simulink library "casper_library_correlator"  (Simulink 8.0)
settings: Solver=ode45  SolverMode=SingleTasking  StartTime=0.0  StopTime=10.0  RelTol=1e-3
values from neighbouring files (symbols this model uses):
  n_bits = eval(get_var('n_bits', 'defaults', defaults, varargin{:}))    [auto_tap_init.m]    (also in baseline_tap_init.m; bi_real_unscr_2x_init.m = get_var('n_bits', 'defaults', defaults, varargin{:}); bi_real_unscr_4x_init.m = get_var('n_bits', 'defaults', defaults, varargin{:}); bit_reverse_init.m = get_var('n_bits',varargin{:}))
libraries: xbsIndex_r4 x1360, casper_library_misc x140, casper_library_multipliers x32, xps_library x8, casper_library_delays x1, casper_library_correlator x1
(part 4 of 14)

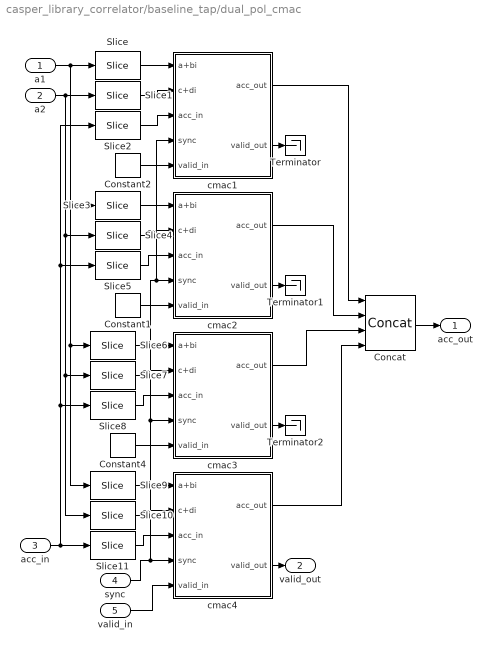
== system casper_library_correlator/baseline_tap/dual_pol_cmac ==
  a1 : Inport
  a2 : Inport  Port=2
  acc_in : Inport  Port=3
  sync : Inport  Port=4
  valid_in : Inport  Port=5
  Concat : xbsIndex_r4/Concat  num_inputs=4  dbl_ovrd=off  block_type=concat
      settings: block_version=9.2.01
  Constant1 : xbsIndex_r4/Constant  const=0  gui_display_data_type=Fixed-point  arith_type=Unsigned  n_bits=1  bin_pt=0  preci_type=Single  exp_width=8  frac_width=24  explicit_period=on  period=1  equ=P=C  opselect=C  inp2=PCIN>>17  opr=+  inp1=P  carry=CIN  dbl_ovrd=off  block_type=constant
      settings: block_version=9.2.01
  Constant2 : xbsIndex_r4/Constant  const=0  gui_display_data_type=Fixed-point  arith_type=Unsigned  n_bits=1  bin_pt=0  preci_type=Single  exp_width=8  frac_width=24  explicit_period=on  period=1  equ=P=C  opselect=C  inp2=PCIN>>17  opr=+  inp1=P  carry=CIN  dbl_ovrd=off  block_type=constant
      settings: block_version=9.2.01
  Constant4 : xbsIndex_r4/Constant  const=0  gui_display_data_type=Fixed-point  arith_type=Unsigned  n_bits=1  bin_pt=0  preci_type=Single  exp_width=8  frac_width=24  explicit_period=on  period=1  equ=P=C  opselect=C  inp2=PCIN>>17  opr=+  inp1=P  carry=CIN  dbl_ovrd=off  block_type=constant
      settings: block_version=9.2.01
  Slice{,1,6,10} (4 alike) : xbsIndex_r4/Slice  nbits=2*n_bits  boolean_output=off  mode=Upper Bit Location + Width  bit1=0  base1=MSB of Input  bit0=0  base0=LSB of Input  dbl_ovrd=off  block_type=slice
      Slice settings: infoedit="Extracts a given range of bits from each input sample and presents it at the output.  The output type is ordinarily unsigned with binary point at zero, but can be Boolean when the slice is one bit wide.<P><P>Hardware notes: In hardware this block costs nothing."  block_version=9.2.01
      Slice1 settings: infoedit="Extracts a given range of bits from each input sample and presents it at the output.  The output type is ordinarily unsigned with binary point at zero, but can be Boolean when the slice is one bit wide.<P><P>Hardware notes: In hardware this block costs nothing."  block_version=9.2.01
      Slice10 settings: block_version=9.2.01
      Slice6 settings: infoedit="Extracts a given range of bits from each input sample and presents it at the output.  The output type is ordinarily unsigned with binary point at zero, but can be Boolean when the slice is one bit wide.<P><P>Hardware notes: In hardware this block costs nothing."  block_version=9.2.01
  Slice11 : xbsIndex_r4/Slice  nbits=2*n_bits_out  boolean_output=off  mode=Upper Bit Location + Width  bit1=-6*n_bits_out  base1=MSB of Input  bit0=0  base0=LSB of Input  dbl_ovrd=off  block_type=slice
      settings: infoedit="Extracts a given range of bits from each input sample and presents it at the output.  The output type is ordinarily unsigned with binary point at zero, but can be Boolean when the slice is one bit wide.<P><P>Hardware notes: In hardware this block costs nothing."  block_version=9.2.01
  Slice2 : xbsIndex_r4/Slice  nbits=2*n_bits_out  boolean_output=off  mode=Upper Bit Location + Width  bit1=0  base1=MSB of Input  bit0=0  base0=LSB of Input  dbl_ovrd=off  block_type=slice
      settings: infoedit="Extracts a given range of bits from each input sample and presents it at the output.  The output type is ordinarily unsigned with binary point at zero, but can be Boolean when the slice is one bit wide.<P><P>Hardware notes: In hardware this block costs nothing."  block_version=9.2.01
  Slice{3..4,7,9} (4 alike) : xbsIndex_r4/Slice  nbits=2*n_bits  boolean_output=off  mode=Upper Bit Location + Width  bit1=-2*n_bits  base1=MSB of Input  bit0=0  base0=LSB of Input  dbl_ovrd=off  block_type=slice
      Slice3 settings: infoedit="Extracts a given range of bits from each input sample and presents it at the output.  The output type is ordinarily unsigned with binary point at zero, but can be Boolean when the slice is one bit wide.<P><P>Hardware notes: In hardware this block costs nothing."  block_version=9.2.01
      Slice4 settings: infoedit="Extracts a given range of bits from each input sample and presents it at the output.  The output type is ordinarily unsigned with binary point at zero, but can be Boolean when the slice is one bit wide.<P><P>Hardware notes: In hardware this block costs nothing."  block_version=9.2.01
      Slice7 settings: infoedit="Extracts a given range of bits from each input sample and presents it at the output.  The output type is ordinarily unsigned with binary point at zero, but can be Boolean when the slice is one bit wide.<P><P>Hardware notes: In hardware this block costs nothing."  block_version=9.2.01
      Slice9 settings: block_version=9.2.01
  Slice5 : xbsIndex_r4/Slice  nbits=2*n_bits_out  boolean_output=off  mode=Upper Bit Location + Width  bit1=-2*n_bits_out  base1=MSB of Input  bit0=0  base0=LSB of Input  dbl_ovrd=off  block_type=slice
      settings: infoedit="Extracts a given range of bits from each input sample and presents it at the output.  The output type is ordinarily unsigned with binary point at zero, but can be Boolean when the slice is one bit wide.<P><P>Hardware notes: In hardware this block costs nothing."  block_version=9.2.01
  Slice8 : xbsIndex_r4/Slice  nbits=2*n_bits_out  boolean_output=off  mode=Upper Bit Location + Width  bit1=-4*n_bits_out  base1=MSB of Input  bit0=0  base0=LSB of Input  dbl_ovrd=off  block_type=slice
      settings: infoedit="Extracts a given range of bits from each input sample and presents it at the output.  The output type is ordinarily unsigned with binary point at zero, but can be Boolean when the slice is one bit wide.<P><P>Hardware notes: In hardware this block costs nothing."  block_version=9.2.01
  Terminator : Terminator
  Terminator1 : Terminator
  Terminator2 : Terminator
  cmac1 : Subsystem  Tag=cmac  AncestorBlock=casper_library_correlator/cmac  mask(cmac){acc_len=128, n_bits_a=4, bin_pt_a=3, n_bits_b=4, bin_pt_b=3, quantization=Truncate, overflow=Wrap, mult_latency=1, add_latency=1, in_latency=0, conv_latency=0, multiplier_implementation=embedded multiplier core}
      mask prompts: acc_len "Number of Accumulations"; n_bits_a "Number of bits 'a'"; bin_pt_a "Binary point 'a'"; n_bits_b "Number of bits 'b'"; bin_pt_b "Binary point 'b'"; quantization "Quantisation"; mult_latency "Multiplier Latency"; add_latency "Adder Latency"; in_latency "Input Latency"; conv_latency "Convert Latency"; multiplier_implementation "Multiplier Implementation"
      mask help: A complex multiply-accumulate block. Full precision.
      mask init: same as casper_library_correlator/dual_pol_cmac/cmac1
      mask TypeOptions quantization: Truncate | Round  (unbiased: +/- Inf) | Round  (unbiased: Even Values)
      mask TypeOptions overflow: Wrap | Saturate | Flag as error
      mask TypeOptions multiplier_implementation: behavioral HDL | standard core | embedded multiplier core
  cmac2 : Subsystem  Tag=cmac  AncestorBlock=casper_library_correlator/cmac  mask(cmac){acc_len=128, n_bits_a=4, bin_pt_a=3, n_bits_b=4, bin_pt_b=3, quantization=Truncate, overflow=Wrap, mult_latency=1, add_latency=1, in_latency=0, conv_latency=0, multiplier_implementation=embedded multiplier core}
      mask prompts: acc_len "Number of Accumulations"; n_bits_a "Number of bits 'a'"; bin_pt_a "Binary point 'a'"; n_bits_b "Number of bits 'b'"; bin_pt_b "Binary point 'b'"; quantization "Quantisation"; mult_latency "Multiplier Latency"; add_latency "Adder Latency"; in_latency "Input Latency"; conv_latency "Convert Latency"; multiplier_implementation "Multiplier Implementation"
      mask help: A complex multiply-accumulate block. Full precision.
      mask init: same as casper_library_correlator/dual_pol_cmac/cmac1
      mask TypeOptions quantization: Truncate | Round  (unbiased: +/- Inf) | Round  (unbiased: Even Values)
      mask TypeOptions overflow: Wrap | Saturate | Flag as error
      mask TypeOptions multiplier_implementation: behavioral HDL | standard core | embedded multiplier core
  cmac3 : Subsystem  Tag=cmac  AncestorBlock=casper_library_correlator/cmac  mask(cmac){acc_len=128, n_bits_a=4, bin_pt_a=3, n_bits_b=4, bin_pt_b=3, quantization=Truncate, overflow=Wrap, mult_latency=1, add_latency=1, in_latency=0, conv_latency=0, multiplier_implementation=embedded multiplier core}
      mask prompts: acc_len "Number of Accumulations"; n_bits_a "Number of bits 'a'"; bin_pt_a "Binary point 'a'"; n_bits_b "Number of bits 'b'"; bin_pt_b "Binary point 'b'"; quantization "Quantisation"; mult_latency "Multiplier Latency"; add_latency "Adder Latency"; in_latency "Input Latency"; conv_latency "Convert Latency"; multiplier_implementation "Multiplier Implementation"
      mask help: A complex multiply-accumulate block. Full precision.
      mask init: same as casper_library_correlator/dual_pol_cmac/cmac1
      mask TypeOptions quantization: Truncate | Round  (unbiased: +/- Inf) | Round  (unbiased: Even Values)
      mask TypeOptions overflow: Wrap | Saturate | Flag as error
      mask TypeOptions multiplier_implementation: behavioral HDL | standard core | embedded multiplier core
  cmac4 : Subsystem  Tag=cmac  AncestorBlock=casper_library_correlator/cmac  mask(cmac){acc_len=128, n_bits_a=4, bin_pt_a=3, n_bits_b=4, bin_pt_b=3, quantization=Truncate, overflow=Wrap, mult_latency=1, add_latency=1, in_latency=0, conv_latency=0, multiplier_implementation=embedded multiplier core}
      mask prompts: acc_len "Number of Accumulations"; n_bits_a "Number of bits 'a'"; bin_pt_a "Binary point 'a'"; n_bits_b "Number of bits 'b'"; bin_pt_b "Binary point 'b'"; quantization "Quantisation"; mult_latency "Multiplier Latency"; add_latency "Adder Latency"; in_latency "Input Latency"; conv_latency "Convert Latency"; multiplier_implementation "Multiplier Implementation"
      mask help: A complex multiply-accumulate block. Full precision.
      mask init: same as casper_library_correlator/dual_pol_cmac/cmac1
      mask TypeOptions quantization: Truncate | Round  (unbiased: +/- Inf) | Round  (unbiased: Even Values)
      mask TypeOptions overflow: Wrap | Saturate | Flag as error
      mask TypeOptions multiplier_implementation: behavioral HDL | standard core | embedded multiplier core
  acc_out : Outport
  valid_out : Outport  Port=2
  wires:
  Constant2/1 -> cmac1/5(valid_in)
  Slice/1 -> cmac1/1(a+bi)
  Slice1/1 -> cmac1/2(c+di)
  Slice2/1 -> cmac1/3(acc_in)
  Slice3/1 -> cmac2/1(a+bi)
  Slice4/1 -> cmac2/2(c+di)
  Slice5/1 -> cmac2/3(acc_in)
  Concat/1 -> acc_out/1
  valid_in/1 -> cmac4/5(valid_in)
  cmac1/2(valid_out) -> Terminator/1
  Constant1/1 -> cmac2/5(valid_in)
  Slice6/1 -> cmac3/1(a+bi)
  Slice7/1 -> cmac3/2(c+di)
  Slice8/1 -> cmac3/3(acc_in)
  Constant4/1 -> cmac3/5(valid_in)
  Slice9/1 -> cmac4/1(a+bi)
  Slice10/1 -> cmac4/2(c+di)
  Slice11/1 -> cmac4/3(acc_in)
  sync/1 -> cmac1/4(sync), cmac2/4(sync), cmac3/4(sync), cmac4/4(sync)
  cmac2/2(valid_out) -> Terminator1/1
  cmac3/2(valid_out) -> Terminator2/1
  cmac4/2(valid_out) -> valid_out/1
  cmac1/1(acc_out) -> Concat/1
  cmac2/1(acc_out) -> Concat/2
  cmac3/1(acc_out) -> Concat/3
  cmac4/1(acc_out) -> Concat/4
  a1/1 -> Slice/1, Slice3/1, Slice6/1, Slice9/1
  a2/1 -> Slice1/1, Slice4/1, Slice7/1, Slice10/1
  acc_in/1 -> Slice11/1, Slice8/1, Slice5/1, Slice2/1

== system casper_library_correlator/cross_multiplier/cvrt0_0_0_imag ==
  din : Inport
  convert : casper_library_misc/convert  bin_pt_in=binary_point_i  n_bits_out=bit_width_o  bin_pt_out=binary_point_o  quantization=Truncate  overflow=Wrap  latency=latency
      settings: AttributesFormatString=|
      | N_7 ==> 4_3
      | truncate, wrap
      | latency = 4
  never : xbsIndex_r4/Constant  const=0  gui_display_data_type=Fixed-point  arith_type=Boolean  n_bits=16  bin_pt=14  preci_type=Single  exp_width=8  frac_width=24  explicit_period=on  period=1  equ=P=C  opselect=C  inp2=PCIN>>17  opr=+  inp1=P  carry=CIN  dbl_ovrd=off  block_type=constant
  dout : Outport
  of : Outport  Port=2
  wires:
  din/1 -> convert/1
  convert/1 -> dout/1
  never/1 -> of/1

== system casper_library_correlator/cross_multiplier/cvrt0_0_0_real ==
  din : Inport
  convert : casper_library_misc/convert  bin_pt_in=binary_point_i  n_bits_out=bit_width_o  bin_pt_out=binary_point_o  quantization=Truncate  overflow=Wrap  latency=latency
      settings: AttributesFormatString=|
      | N_7 ==> 4_3
      | truncate, wrap
      | latency = 4
  never : xbsIndex_r4/Constant  const=0  gui_display_data_type=Fixed-point  arith_type=Boolean  n_bits=16  bin_pt=14  preci_type=Single  exp_width=8  frac_width=24  explicit_period=on  period=1  equ=P=C  opselect=C  inp2=PCIN>>17  opr=+  inp1=P  carry=CIN  dbl_ovrd=off  block_type=constant
  dout : Outport
  of : Outport  Port=2
  wires:
  din/1 -> convert/1
  convert/1 -> dout/1
  never/1 -> of/1

== system casper_library_correlator/cross_multiplier/cvrt0_0_1_imag ==
  din : Inport
  convert : casper_library_misc/convert  bin_pt_in=binary_point_i  n_bits_out=bit_width_o  bin_pt_out=binary_point_o  quantization=Truncate  overflow=Wrap  latency=latency
      settings: AttributesFormatString=|
      | N_7 ==> 4_3
      | truncate, wrap
      | latency = 4
  never : xbsIndex_r4/Constant  const=0  gui_display_data_type=Fixed-point  arith_type=Boolean  n_bits=16  bin_pt=14  preci_type=Single  exp_width=8  frac_width=24  explicit_period=on  period=1  equ=P=C  opselect=C  inp2=PCIN>>17  opr=+  inp1=P  carry=CIN  dbl_ovrd=off  block_type=constant
  dout : Outport
  of : Outport  Port=2
  wires:
  din/1 -> convert/1
  convert/1 -> dout/1
  never/1 -> of/1

== system casper_library_correlator/cross_multiplier/cvrt0_0_1_real ==
  din : Inport
  convert : casper_library_misc/convert  bin_pt_in=binary_point_i  n_bits_out=bit_width_o  bin_pt_out=binary_point_o  quantization=Truncate  overflow=Wrap  latency=latency
      settings: AttributesFormatString=|
      | N_7 ==> 4_3
      | truncate, wrap
      | latency = 4
  never : xbsIndex_r4/Constant  const=0  gui_display_data_type=Fixed-point  arith_type=Boolean  n_bits=16  bin_pt=14  preci_type=Single  exp_width=8  frac_width=24  explicit_period=on  period=1  equ=P=C  opselect=C  inp2=PCIN>>17  opr=+  inp1=P  carry=CIN  dbl_ovrd=off  block_type=constant
  dout : Outport
  of : Outport  Port=2
  wires:
  din/1 -> convert/1
  convert/1 -> dout/1
  never/1 -> of/1

== system casper_library_correlator/cross_multiplier/cvrt1_0_0_imag ==
  din : Inport
  convert : casper_library_misc/convert  bin_pt_in=binary_point_i  n_bits_out=bit_width_o  bin_pt_out=binary_point_o  quantization=Truncate  overflow=Wrap  latency=latency
      settings: AttributesFormatString=|
      | N_7 ==> 4_3
      | truncate, wrap
      | latency = 4
  never : xbsIndex_r4/Constant  const=0  gui_display_data_type=Fixed-point  arith_type=Boolean  n_bits=16  bin_pt=14  preci_type=Single  exp_width=8  frac_width=24  explicit_period=on  period=1  equ=P=C  opselect=C  inp2=PCIN>>17  opr=+  inp1=P  carry=CIN  dbl_ovrd=off  block_type=constant
  dout : Outport
  of : Outport  Port=2
  wires:
  din/1 -> convert/1
  convert/1 -> dout/1
  never/1 -> of/1

== system casper_library_correlator/cross_multiplier/cvrt1_0_0_real ==
  din : Inport
  convert : casper_library_misc/convert  bin_pt_in=binary_point_i  n_bits_out=bit_width_o  bin_pt_out=binary_point_o  quantization=Truncate  overflow=Wrap  latency=latency
      settings: AttributesFormatString=|
      | N_7 ==> 4_3
      | truncate, wrap
      | latency = 4
  never : xbsIndex_r4/Constant  const=0  gui_display_data_type=Fixed-point  arith_type=Boolean  n_bits=16  bin_pt=14  preci_type=Single  exp_width=8  frac_width=24  explicit_period=on  period=1  equ=P=C  opselect=C  inp2=PCIN>>17  opr=+  inp1=P  carry=CIN  dbl_ovrd=off  block_type=constant
  dout : Outport
  of : Outport  Port=2
  wires:
  din/1 -> convert/1
  convert/1 -> dout/1
  never/1 -> of/1

== system casper_library_correlator/cross_multiplier/cvrt1_0_1_imag ==
  din : Inport
  convert : casper_library_misc/convert  bin_pt_in=binary_point_i  n_bits_out=bit_width_o  bin_pt_out=binary_point_o  quantization=Truncate  overflow=Wrap  latency=latency
      settings: AttributesFormatString=|
      | N_7 ==> 4_3
      | truncate, wrap
      | latency = 4
  never : xbsIndex_r4/Constant  const=0  gui_display_data_type=Fixed-point  arith_type=Boolean  n_bits=16  bin_pt=14  preci_type=Single  exp_width=8  frac_width=24  explicit_period=on  period=1  equ=P=C  opselect=C  inp2=PCIN>>17  opr=+  inp1=P  carry=CIN  dbl_ovrd=off  block_type=constant
  dout : Outport
  of : Outport  Port=2
  wires:
  din/1 -> convert/1
  convert/1 -> dout/1
  never/1 -> of/1

== system casper_library_correlator/cross_multiplier/cvrt1_0_1_real ==
  din : Inport
  convert : casper_library_misc/convert  bin_pt_in=binary_point_i  n_bits_out=bit_width_o  bin_pt_out=binary_point_o  quantization=Truncate  overflow=Wrap  latency=latency
      settings: AttributesFormatString=|
      | N_7 ==> 4_3
      | truncate, wrap
      | latency = 4
  never : xbsIndex_r4/Constant  const=0  gui_display_data_type=Fixed-point  arith_type=Boolean  n_bits=16  bin_pt=14  preci_type=Single  exp_width=8  frac_width=24  explicit_period=on  period=1  equ=P=C  opselect=C  inp2=PCIN>>17  opr=+  inp1=P  carry=CIN  dbl_ovrd=off  block_type=constant
  dout : Outport
  of : Outport  Port=2
  wires:
  din/1 -> convert/1
  convert/1 -> dout/1
  never/1 -> of/1

== system casper_library_correlator/cross_multiplier/cvrt1_1_0_imag ==
  din : Inport
  convert : casper_library_misc/convert  bin_pt_in=binary_point_i  n_bits_out=bit_width_o  bin_pt_out=binary_point_o  quantization=Truncate  overflow=Wrap  latency=latency
      settings: AttributesFormatString=|
      | N_7 ==> 4_3
      | truncate, wrap
      | latency = 4
  never : xbsIndex_r4/Constant  const=0  gui_display_data_type=Fixed-point  arith_type=Boolean  n_bits=16  bin_pt=14  preci_type=Single  exp_width=8  frac_width=24  explicit_period=on  period=1  equ=P=C  opselect=C  inp2=PCIN>>17  opr=+  inp1=P  carry=CIN  dbl_ovrd=off  block_type=constant
  dout : Outport
  of : Outport  Port=2
  wires:
  din/1 -> convert/1
  convert/1 -> dout/1
  never/1 -> of/1

== system casper_library_correlator/cross_multiplier/cvrt1_1_0_real ==
  din : Inport
  convert : casper_library_misc/convert  bin_pt_in=binary_point_i  n_bits_out=bit_width_o  bin_pt_out=binary_point_o  quantization=Truncate  overflow=Wrap  latency=latency
      settings: AttributesFormatString=|
      | N_7 ==> 4_3
      | truncate, wrap
      | latency = 4
  never : xbsIndex_r4/Constant  const=0  gui_display_data_type=Fixed-point  arith_type=Boolean  n_bits=16  bin_pt=14  preci_type=Single  exp_width=8  frac_width=24  explicit_period=on  period=1  equ=P=C  opselect=C  inp2=PCIN>>17  opr=+  inp1=P  carry=CIN  dbl_ovrd=off  block_type=constant
  dout : Outport
  of : Outport  Port=2
  wires:
  din/1 -> convert/1
  convert/1 -> dout/1
  never/1 -> of/1

== system casper_library_correlator/cross_multiplier/cvrt1_1_1_imag ==
  din : Inport
  convert : casper_library_misc/convert  bin_pt_in=binary_point_i  n_bits_out=bit_width_o  bin_pt_out=binary_point_o  quantization=Truncate  overflow=Wrap  latency=latency
      settings: AttributesFormatString=|
      | N_7 ==> 4_3
      | truncate, wrap
      | latency = 4
  never : xbsIndex_r4/Constant  const=0  gui_display_data_type=Fixed-point  arith_type=Boolean  n_bits=16  bin_pt=14  preci_type=Single  exp_width=8  frac_width=24  explicit_period=on  period=1  equ=P=C  opselect=C  inp2=PCIN>>17  opr=+  inp1=P  carry=CIN  dbl_ovrd=off  block_type=constant
  dout : Outport
  of : Outport  Port=2
  wires:
  din/1 -> convert/1
  convert/1 -> dout/1
  never/1 -> of/1

== system casper_library_correlator/cross_multiplier/cvrt1_1_1_real ==
  din : Inport
  convert : casper_library_misc/convert  bin_pt_in=binary_point_i  n_bits_out=bit_width_o  bin_pt_out=binary_point_o  quantization=Truncate  overflow=Wrap  latency=latency
      settings: AttributesFormatString=|
      | N_7 ==> 4_3
      | truncate, wrap
      | latency = 4
  never : xbsIndex_r4/Constant  const=0  gui_display_data_type=Fixed-point  arith_type=Boolean  n_bits=16  bin_pt=14  preci_type=Single  exp_width=8  frac_width=24  explicit_period=on  period=1  equ=P=C  opselect=C  inp2=PCIN>>17  opr=+  inp1=P  carry=CIN  dbl_ovrd=off  block_type=constant
  dout : Outport
  of : Outport  Port=2
  wires:
  din/1 -> convert/1
  convert/1 -> dout/1
  never/1 -> of/1

== system casper_library_correlator/cross_multiplier/cvrt1_2_0_imag ==
  din : Inport
  convert : casper_library_misc/convert  bin_pt_in=binary_point_i  n_bits_out=bit_width_o  bin_pt_out=binary_point_o  quantization=Truncate  overflow=Wrap  latency=latency
      settings: AttributesFormatString=|
      | N_7 ==> 4_3
      | truncate, wrap
      | latency = 4
  never : xbsIndex_r4/Constant  const=0  gui_display_data_type=Fixed-point  arith_type=Boolean  n_bits=16  bin_pt=14  preci_type=Single  exp_width=8  frac_width=24  explicit_period=on  period=1  equ=P=C  opselect=C  inp2=PCIN>>17  opr=+  inp1=P  carry=CIN  dbl_ovrd=off  block_type=constant
  dout : Outport
  of : Outport  Port=2
  wires:
  din/1 -> convert/1
  convert/1 -> dout/1
  never/1 -> of/1

== system casper_library_correlator/cross_multiplier/cvrt1_2_0_real ==
  din : Inport
  convert : casper_library_misc/convert  bin_pt_in=binary_point_i  n_bits_out=bit_width_o  bin_pt_out=binary_point_o  quantization=Truncate  overflow=Wrap  latency=latency
      settings: AttributesFormatString=|
      | N_7 ==> 4_3
      | truncate, wrap
      | latency = 4
  never : xbsIndex_r4/Constant  const=0  gui_display_data_type=Fixed-point  arith_type=Boolean  n_bits=16  bin_pt=14  preci_type=Single  exp_width=8  frac_width=24  explicit_period=on  period=1  equ=P=C  opselect=C  inp2=PCIN>>17  opr=+  inp1=P  carry=CIN  dbl_ovrd=off  block_type=constant
  dout : Outport
  of : Outport  Port=2
  wires:
  din/1 -> convert/1
  convert/1 -> dout/1
  never/1 -> of/1

== system casper_library_correlator/cross_multiplier/cvrt1_2_1_imag ==
  din : Inport
  convert : casper_library_misc/convert  bin_pt_in=binary_point_i  n_bits_out=bit_width_o  bin_pt_out=binary_point_o  quantization=Truncate  overflow=Wrap  latency=latency
      settings: AttributesFormatString=|
      | N_7 ==> 4_3
      | truncate, wrap
      | latency = 4
  never : xbsIndex_r4/Constant  const=0  gui_display_data_type=Fixed-point  arith_type=Boolean  n_bits=16  bin_pt=14  preci_type=Single  exp_width=8  frac_width=24  explicit_period=on  period=1  equ=P=C  opselect=C  inp2=PCIN>>17  opr=+  inp1=P  carry=CIN  dbl_ovrd=off  block_type=constant
  dout : Outport
  of : Outport  Port=2
  wires:
  din/1 -> convert/1
  convert/1 -> dout/1
  never/1 -> of/1

== system casper_library_correlator/cross_multiplier/cvrt1_2_1_real ==
  din : Inport
  convert : casper_library_misc/convert  bin_pt_in=binary_point_i  n_bits_out=bit_width_o  bin_pt_out=binary_point_o  quantization=Truncate  overflow=Wrap  latency=latency
      settings: AttributesFormatString=|
      | N_7 ==> 4_3
      | truncate, wrap
      | latency = 4
  never : xbsIndex_r4/Constant  const=0  gui_display_data_type=Fixed-point  arith_type=Boolean  n_bits=16  bin_pt=14  preci_type=Single  exp_width=8  frac_width=24  explicit_period=on  period=1  equ=P=C  opselect=C  inp2=PCIN>>17  opr=+  inp1=P  carry=CIN  dbl_ovrd=off  block_type=constant
  dout : Outport
  of : Outport  Port=2
  wires:
  din/1 -> convert/1
  convert/1 -> dout/1
  never/1 -> of/1

== system casper_library_correlator/cross_multiplier/cvrt2_0_0_imag ==
  din : Inport
  convert : casper_library_misc/convert  bin_pt_in=binary_point_i  n_bits_out=bit_width_o  bin_pt_out=binary_point_o  quantization=Truncate  overflow=Wrap  latency=latency
      settings: AttributesFormatString=|
      | N_7 ==> 4_3
      | truncate, wrap
      | latency = 4
  never : xbsIndex_r4/Constant  const=0  gui_display_data_type=Fixed-point  arith_type=Boolean  n_bits=16  bin_pt=14  preci_type=Single  exp_width=8  frac_width=24  explicit_period=on  period=1  equ=P=C  opselect=C  inp2=PCIN>>17  opr=+  inp1=P  carry=CIN  dbl_ovrd=off  block_type=constant
  dout : Outport
  of : Outport  Port=2
  wires:
  din/1 -> convert/1
  convert/1 -> dout/1
  never/1 -> of/1

== system casper_library_correlator/cross_multiplier/cvrt2_0_0_real ==
  din : Inport
  convert : casper_library_misc/convert  bin_pt_in=binary_point_i  n_bits_out=bit_width_o  bin_pt_out=binary_point_o  quantization=Truncate  overflow=Wrap  latency=latency
      settings: AttributesFormatString=|
      | N_7 ==> 4_3
      | truncate, wrap
      | latency = 4
  never : xbsIndex_r4/Constant  const=0  gui_display_data_type=Fixed-point  arith_type=Boolean  n_bits=16  bin_pt=14  preci_type=Single  exp_width=8  frac_width=24  explicit_period=on  period=1  equ=P=C  opselect=C  inp2=PCIN>>17  opr=+  inp1=P  carry=CIN  dbl_ovrd=off  block_type=constant
  dout : Outport
  of : Outport  Port=2
  wires:
  din/1 -> convert/1
  convert/1 -> dout/1
  never/1 -> of/1

== system casper_library_correlator/cross_multiplier/cvrt2_0_1_imag ==
  din : Inport
  convert : casper_library_misc/convert  bin_pt_in=binary_point_i  n_bits_out=bit_width_o  bin_pt_out=binary_point_o  quantization=Truncate  overflow=Wrap  latency=latency
      settings: AttributesFormatString=|
      | N_7 ==> 4_3
      | truncate, wrap
      | latency = 4
  never : xbsIndex_r4/Constant  const=0  gui_display_data_type=Fixed-point  arith_type=Boolean  n_bits=16  bin_pt=14  preci_type=Single  exp_width=8  frac_width=24  explicit_period=on  period=1  equ=P=C  opselect=C  inp2=PCIN>>17  opr=+  inp1=P  carry=CIN  dbl_ovrd=off  block_type=constant
  dout : Outport
  of : Outport  Port=2
  wires:
  din/1 -> convert/1
  convert/1 -> dout/1
  never/1 -> of/1

== system casper_library_correlator/cross_multiplier/cvrt2_0_1_real ==
  din : Inport
  convert : casper_library_misc/convert  bin_pt_in=binary_point_i  n_bits_out=bit_width_o  bin_pt_out=binary_point_o  quantization=Truncate  overflow=Wrap  latency=latency
      settings: AttributesFormatString=|
      | N_7 ==> 4_3
      | truncate, wrap
      | latency = 4
  never : xbsIndex_r4/Constant  const=0  gui_display_data_type=Fixed-point  arith_type=Boolean  n_bits=16  bin_pt=14  preci_type=Single  exp_width=8  frac_width=24  explicit_period=on  period=1  equ=P=C  opselect=C  inp2=PCIN>>17  opr=+  inp1=P  carry=CIN  dbl_ovrd=off  block_type=constant
  dout : Outport
  of : Outport  Port=2
  wires:
  din/1 -> convert/1
  convert/1 -> dout/1
  never/1 -> of/1

== system casper_library_correlator/cross_multiplier/cvrt2_1_0_imag ==
  din : Inport
  convert : casper_library_misc/convert  bin_pt_in=binary_point_i  n_bits_out=bit_width_o  bin_pt_out=binary_point_o  quantization=Truncate  overflow=Wrap  latency=latency
      settings: AttributesFormatString=|
      | N_7 ==> 4_3
      | truncate, wrap
      | latency = 4
  never : xbsIndex_r4/Constant  const=0  gui_display_data_type=Fixed-point  arith_type=Boolean  n_bits=16  bin_pt=14  preci_type=Single  exp_width=8  frac_width=24  explicit_period=on  period=1  equ=P=C  opselect=C  inp2=PCIN>>17  opr=+  inp1=P  carry=CIN  dbl_ovrd=off  block_type=constant
  dout : Outport
  of : Outport  Port=2
  wires:
  din/1 -> convert/1
  convert/1 -> dout/1
  never/1 -> of/1

== system casper_library_correlator/cross_multiplier/cvrt2_1_0_real ==
  din : Inport
  convert : casper_library_misc/convert  bin_pt_in=binary_point_i  n_bits_out=bit_width_o  bin_pt_out=binary_point_o  quantization=Truncate  overflow=Wrap  latency=latency
      settings: AttributesFormatString=|
      | N_7 ==> 4_3
      | truncate, wrap
      | latency = 4
  never : xbsIndex_r4/Constant  const=0  gui_display_data_type=Fixed-point  arith_type=Boolean  n_bits=16  bin_pt=14  preci_type=Single  exp_width=8  frac_width=24  explicit_period=on  period=1  equ=P=C  opselect=C  inp2=PCIN>>17  opr=+  inp1=P  carry=CIN  dbl_ovrd=off  block_type=constant
  dout : Outport
  of : Outport  Port=2
  wires:
  din/1 -> convert/1
  convert/1 -> dout/1
  never/1 -> of/1

== system casper_library_correlator/cross_multiplier/cvrt2_1_1_imag ==
  din : Inport
  convert : casper_library_misc/convert  bin_pt_in=binary_point_i  n_bits_out=bit_width_o  bin_pt_out=binary_point_o  quantization=Truncate  overflow=Wrap  latency=latency
      settings: AttributesFormatString=|
      | N_7 ==> 4_3
      | truncate, wrap
      | latency = 4
  never : xbsIndex_r4/Constant  const=0  gui_display_data_type=Fixed-point  arith_type=Boolean  n_bits=16  bin_pt=14  preci_type=Single  exp_width=8  frac_width=24  explicit_period=on  period=1  equ=P=C  opselect=C  inp2=PCIN>>17  opr=+  inp1=P  carry=CIN  dbl_ovrd=off  block_type=constant
  dout : Outport
  of : Outport  Port=2
  wires:
  din/1 -> convert/1
  convert/1 -> dout/1
  never/1 -> of/1

== system casper_library_correlator/cross_multiplier/cvrt2_1_1_real ==
  din : Inport
  convert : casper_library_misc/convert  bin_pt_in=binary_point_i  n_bits_out=bit_width_o  bin_pt_out=binary_point_o  quantization=Truncate  overflow=Wrap  latency=latency
      settings: AttributesFormatString=|
      | N_7 ==> 4_3
      | truncate, wrap
      | latency = 4
  never : xbsIndex_r4/Constant  const=0  gui_display_data_type=Fixed-point  arith_type=Boolean  n_bits=16  bin_pt=14  preci_type=Single  exp_width=8  frac_width=24  explicit_period=on  period=1  equ=P=C  opselect=C  inp2=PCIN>>17  opr=+  inp1=P  carry=CIN  dbl_ovrd=off  block_type=constant
  dout : Outport
  of : Outport  Port=2
  wires:
  din/1 -> convert/1
  convert/1 -> dout/1
  never/1 -> of/1

== system casper_library_correlator/cross_multiplier/cvrt2_2_0_imag ==
  din : Inport
  convert : casper_library_misc/convert  bin_pt_in=binary_point_i  n_bits_out=bit_width_o  bin_pt_out=binary_point_o  quantization=Truncate  overflow=Wrap  latency=latency
      settings: AttributesFormatString=|
      | N_7 ==> 4_3
      | truncate, wrap
      | latency = 4
  never : xbsIndex_r4/Constant  const=0  gui_display_data_type=Fixed-point  arith_type=Boolean  n_bits=16  bin_pt=14  preci_type=Single  exp_width=8  frac_width=24  explicit_period=on  period=1  equ=P=C  opselect=C  inp2=PCIN>>17  opr=+  inp1=P  carry=CIN  dbl_ovrd=off  block_type=constant
  dout : Outport
  of : Outport  Port=2
  wires:
  din/1 -> convert/1
  convert/1 -> dout/1
  never/1 -> of/1

== system casper_library_correlator/cross_multiplier/cvrt2_2_0_real ==
  din : Inport
  convert : casper_library_misc/convert  bin_pt_in=binary_point_i  n_bits_out=bit_width_o  bin_pt_out=binary_point_o  quantization=Truncate  overflow=Wrap  latency=latency
      settings: AttributesFormatString=|
      | N_7 ==> 4_3
      | truncate, wrap
      | latency = 4
  never : xbsIndex_r4/Constant  const=0  gui_display_data_type=Fixed-point  arith_type=Boolean  n_bits=16  bin_pt=14  preci_type=Single  exp_width=8  frac_width=24  explicit_period=on  period=1  equ=P=C  opselect=C  inp2=PCIN>>17  opr=+  inp1=P  carry=CIN  dbl_ovrd=off  block_type=constant
  dout : Outport
  of : Outport  Port=2
  wires:
  din/1 -> convert/1
  convert/1 -> dout/1
  never/1 -> of/1

== system casper_library_correlator/cross_multiplier/cvrt2_2_1_imag ==
  din : Inport
  convert : casper_library_misc/convert  bin_pt_in=binary_point_i  n_bits_out=bit_width_o  bin_pt_out=binary_point_o  quantization=Truncate  overflow=Wrap  latency=latency
      settings: AttributesFormatString=|
      | N_7 ==> 4_3
      | truncate, wrap
      | latency = 4
  never : xbsIndex_r4/Constant  const=0  gui_display_data_type=Fixed-point  arith_type=Boolean  n_bits=16  bin_pt=14  preci_type=Single  exp_width=8  frac_width=24  explicit_period=on  period=1  equ=P=C  opselect=C  inp2=PCIN>>17  opr=+  inp1=P  carry=CIN  dbl_ovrd=off  block_type=constant
  dout : Outport
  of : Outport  Port=2
  wires:
  din/1 -> convert/1
  convert/1 -> dout/1
  never/1 -> of/1

== system casper_library_correlator/cross_multiplier/cvrt2_2_1_real ==
  din : Inport
  convert : casper_library_misc/convert  bin_pt_in=binary_point_i  n_bits_out=bit_width_o  bin_pt_out=binary_point_o  quantization=Truncate  overflow=Wrap  latency=latency
      settings: AttributesFormatString=|
      | N_7 ==> 4_3
      | truncate, wrap
      | latency = 4
  never : xbsIndex_r4/Constant  const=0  gui_display_data_type=Fixed-point  arith_type=Boolean  n_bits=16  bin_pt=14  preci_type=Single  exp_width=8  frac_width=24  explicit_period=on  period=1  equ=P=C  opselect=C  inp2=PCIN>>17  opr=+  inp1=P  carry=CIN  dbl_ovrd=off  block_type=constant
  dout : Outport
  of : Outport  Port=2
  wires:
  din/1 -> convert/1
  convert/1 -> dout/1
  never/1 -> of/1

== system casper_library_correlator/cross_multiplier/cvrt2_3_0_imag ==
  din : Inport
  convert : casper_library_misc/convert  bin_pt_in=binary_point_i  n_bits_out=bit_width_o  bin_pt_out=binary_point_o  quantization=Truncate  overflow=Wrap  latency=latency
      settings: AttributesFormatString=|
      | N_7 ==> 4_3
      | truncate, wrap
      | latency = 4
  never : xbsIndex_r4/Constant  const=0  gui_display_data_type=Fixed-point  arith_type=Boolean  n_bits=16  bin_pt=14  preci_type=Single  exp_width=8  frac_width=24  explicit_period=on  period=1  equ=P=C  opselect=C  inp2=PCIN>>17  opr=+  inp1=P  carry=CIN  dbl_ovrd=off  block_type=constant
  dout : Outport
  of : Outport  Port=2
  wires:
  din/1 -> convert/1
  convert/1 -> dout/1
  never/1 -> of/1

== system casper_library_correlator/cross_multiplier/cvrt2_3_0_real ==
  din : Inport
  convert : casper_library_misc/convert  bin_pt_in=binary_point_i  n_bits_out=bit_width_o  bin_pt_out=binary_point_o  quantization=Truncate  overflow=Wrap  latency=latency
      settings: AttributesFormatString=|
      | N_7 ==> 4_3
      | truncate, wrap
      | latency = 4
  never : xbsIndex_r4/Constant  const=0  gui_display_data_type=Fixed-point  arith_type=Boolean  n_bits=16  bin_pt=14  preci_type=Single  exp_width=8  frac_width=24  explicit_period=on  period=1  equ=P=C  opselect=C  inp2=PCIN>>17  opr=+  inp1=P  carry=CIN  dbl_ovrd=off  block_type=constant
  dout : Outport
  of : Outport  Port=2
  wires:
  din/1 -> convert/1
  convert/1 -> dout/1
  never/1 -> of/1

== system casper_library_correlator/cross_multiplier/cvrt2_3_1_imag ==
  din : Inport
  convert : casper_library_misc/convert  bin_pt_in=binary_point_i  n_bits_out=bit_width_o  bin_pt_out=binary_point_o  quantization=Truncate  overflow=Wrap  latency=latency
      settings: AttributesFormatString=|
      | N_7 ==> 4_3
      | truncate, wrap
      | latency = 4
  never : xbsIndex_r4/Constant  const=0  gui_display_data_type=Fixed-point  arith_type=Boolean  n_bits=16  bin_pt=14  preci_type=Single  exp_width=8  frac_width=24  explicit_period=on  period=1  equ=P=C  opselect=C  inp2=PCIN>>17  opr=+  inp1=P  carry=CIN  dbl_ovrd=off  block_type=constant
  dout : Outport
  of : Outport  Port=2
  wires:
  din/1 -> convert/1
  convert/1 -> dout/1
  never/1 -> of/1

== system casper_library_correlator/cross_multiplier/cvrt2_3_1_real ==
  din : Inport
  convert : casper_library_misc/convert  bin_pt_in=binary_point_i  n_bits_out=bit_width_o  bin_pt_out=binary_point_o  quantization=Truncate  overflow=Wrap  latency=latency
      settings: AttributesFormatString=|
      | N_7 ==> 4_3
      | truncate, wrap
      | latency = 4
  never : xbsIndex_r4/Constant  const=0  gui_display_data_type=Fixed-point  arith_type=Boolean  n_bits=16  bin_pt=14  preci_type=Single  exp_width=8  frac_width=24  explicit_period=on  period=1  equ=P=C  opselect=C  inp2=PCIN>>17  opr=+  inp1=P  carry=CIN  dbl_ovrd=off  block_type=constant
  dout : Outport
  of : Outport  Port=2
  wires:
  din/1 -> convert/1
  convert/1 -> dout/1
  never/1 -> of/1

== system casper_library_correlator/cross_multiplier/cvrt2_4_0_imag ==
  din : Inport
  convert : casper_library_misc/convert  bin_pt_in=binary_point_i  n_bits_out=bit_width_o  bin_pt_out=binary_point_o  quantization=Truncate  overflow=Wrap  latency=latency
      settings: AttributesFormatString=|
      | N_7 ==> 4_3
      | truncate, wrap
      | latency = 4
  never : xbsIndex_r4/Constant  const=0  gui_display_data_type=Fixed-point  arith_type=Boolean  n_bits=16  bin_pt=14  preci_type=Single  exp_width=8  frac_width=24  explicit_period=on  period=1  equ=P=C  opselect=C  inp2=PCIN>>17  opr=+  inp1=P  carry=CIN  dbl_ovrd=off  block_type=constant
  dout : Outport
  of : Outport  Port=2
  wires:
  din/1 -> convert/1
  convert/1 -> dout/1
  never/1 -> of/1

== system casper_library_correlator/cross_multiplier/cvrt2_4_0_real ==
  din : Inport
  convert : casper_library_misc/convert  bin_pt_in=binary_point_i  n_bits_out=bit_width_o  bin_pt_out=binary_point_o  quantization=Truncate  overflow=Wrap  latency=latency
      settings: AttributesFormatString=|
      | N_7 ==> 4_3
      | truncate, wrap
      | latency = 4
  never : xbsIndex_r4/Constant  const=0  gui_display_data_type=Fixed-point  arith_type=Boolean  n_bits=16  bin_pt=14  preci_type=Single  exp_width=8  frac_width=24  explicit_period=on  period=1  equ=P=C  opselect=C  inp2=PCIN>>17  opr=+  inp1=P  carry=CIN  dbl_ovrd=off  block_type=constant
  dout : Outport
  of : Outport  Port=2
  wires:
  din/1 -> convert/1
  convert/1 -> dout/1
  never/1 -> of/1

== system casper_library_correlator/cross_multiplier/cvrt2_4_1_imag ==
  din : Inport
  convert : casper_library_misc/convert  bin_pt_in=binary_point_i  n_bits_out=bit_width_o  bin_pt_out=binary_point_o  quantization=Truncate  overflow=Wrap  latency=latency
      settings: AttributesFormatString=|
      | N_7 ==> 4_3
      | truncate, wrap
      | latency = 4
  never : xbsIndex_r4/Constant  const=0  gui_display_data_type=Fixed-point  arith_type=Boolean  n_bits=16  bin_pt=14  preci_type=Single  exp_width=8  frac_width=24  explicit_period=on  period=1  equ=P=C  opselect=C  inp2=PCIN>>17  opr=+  inp1=P  carry=CIN  dbl_ovrd=off  block_type=constant
  dout : Outport
  of : Outport  Port=2
  wires:
  din/1 -> convert/1
  convert/1 -> dout/1
  never/1 -> of/1

== system casper_library_correlator/cross_multiplier/cvrt2_4_1_real ==
  din : Inport
  convert : casper_library_misc/convert  bin_pt_in=binary_point_i  n_bits_out=bit_width_o  bin_pt_out=binary_point_o  quantization=Truncate  overflow=Wrap  latency=latency
      settings: AttributesFormatString=|
      | N_7 ==> 4_3
      | truncate, wrap
      | latency = 4
  never : xbsIndex_r4/Constant  const=0  gui_display_data_type=Fixed-point  arith_type=Boolean  n_bits=16  bin_pt=14  preci_type=Single  exp_width=8  frac_width=24  explicit_period=on  period=1  equ=P=C  opselect=C  inp2=PCIN>>17  opr=+  inp1=P  carry=CIN  dbl_ovrd=off  block_type=constant
  dout : Outport
  of : Outport  Port=2
  wires:
  din/1 -> convert/1
  convert/1 -> dout/1
  never/1 -> of/1

== system casper_library_correlator/cross_multiplier/cvrt3_0_0_imag ==
  din : Inport
  convert : casper_library_misc/convert  bin_pt_in=binary_point_i  n_bits_out=bit_width_o  bin_pt_out=binary_point_o  quantization=Truncate  overflow=Wrap  latency=latency
      settings: AttributesFormatString=|
      | N_7 ==> 4_3
      | truncate, wrap
      | latency = 4
  never : xbsIndex_r4/Constant  const=0  gui_display_data_type=Fixed-point  arith_type=Boolean  n_bits=16  bin_pt=14  preci_type=Single  exp_width=8  frac_width=24  explicit_period=on  period=1  equ=P=C  opselect=C  inp2=PCIN>>17  opr=+  inp1=P  carry=CIN  dbl_ovrd=off  block_type=constant
  dout : Outport
  of : Outport  Port=2
  wires:
  din/1 -> convert/1
  convert/1 -> dout/1
  never/1 -> of/1

== system casper_library_correlator/cross_multiplier/cvrt3_0_0_real ==
  din : Inport
  convert : casper_library_misc/convert  bin_pt_in=binary_point_i  n_bits_out=bit_width_o  bin_pt_out=binary_point_o  quantization=Truncate  overflow=Wrap  latency=latency
      settings: AttributesFormatString=|
      | N_7 ==> 4_3
      | truncate, wrap
      | latency = 4
  never : xbsIndex_r4/Constant  const=0  gui_display_data_type=Fixed-point  arith_type=Boolean  n_bits=16  bin_pt=14  preci_type=Single  exp_width=8  frac_width=24  explicit_period=on  period=1  equ=P=C  opselect=C  inp2=PCIN>>17  opr=+  inp1=P  carry=CIN  dbl_ovrd=off  block_type=constant
  dout : Outport
  of : Outport  Port=2
  wires:
  din/1 -> convert/1
  convert/1 -> dout/1
  never/1 -> of/1

== system casper_library_correlator/cross_multiplier/cvrt3_0_1_imag ==
  din : Inport
  convert : casper_library_misc/convert  bin_pt_in=binary_point_i  n_bits_out=bit_width_o  bin_pt_out=binary_point_o  quantization=Truncate  overflow=Wrap  latency=latency
      settings: AttributesFormatString=|
      | N_7 ==> 4_3
      | truncate, wrap
      | latency = 4
  never : xbsIndex_r4/Constant  const=0  gui_display_data_type=Fixed-point  arith_type=Boolean  n_bits=16  bin_pt=14  preci_type=Single  exp_width=8  frac_width=24  explicit_period=on  period=1  equ=P=C  opselect=C  inp2=PCIN>>17  opr=+  inp1=P  carry=CIN  dbl_ovrd=off  block_type=constant
  dout : Outport
  of : Outport  Port=2
  wires:
  din/1 -> convert/1
  convert/1 -> dout/1
  never/1 -> of/1

== system casper_library_correlator/cross_multiplier/cvrt3_0_1_real ==
  din : Inport
  convert : casper_library_misc/convert  bin_pt_in=binary_point_i  n_bits_out=bit_width_o  bin_pt_out=binary_point_o  quantization=Truncate  overflow=Wrap  latency=latency
      settings: AttributesFormatString=|
      | N_7 ==> 4_3
      | truncate, wrap
      | latency = 4
  never : xbsIndex_r4/Constant  const=0  gui_display_data_type=Fixed-point  arith_type=Boolean  n_bits=16  bin_pt=14  preci_type=Single  exp_width=8  frac_width=24  explicit_period=on  period=1  equ=P=C  opselect=C  inp2=PCIN>>17  opr=+  inp1=P  carry=CIN  dbl_ovrd=off  block_type=constant
  dout : Outport
  of : Outport  Port=2
  wires:
  din/1 -> convert/1
  convert/1 -> dout/1
  never/1 -> of/1

== system casper_library_correlator/cross_multiplier/cvrt3_1_0_imag ==
  din : Inport
  convert : casper_library_misc/convert  bin_pt_in=binary_point_i  n_bits_out=bit_width_o  bin_pt_out=binary_point_o  quantization=Truncate  overflow=Wrap  latency=latency
      settings: AttributesFormatString=|
      | N_7 ==> 4_3
      | truncate, wrap
      | latency = 4
  never : xbsIndex_r4/Constant  const=0  gui_display_data_type=Fixed-point  arith_type=Boolean  n_bits=16  bin_pt=14  preci_type=Single  exp_width=8  frac_width=24  explicit_period=on  period=1  equ=P=C  opselect=C  inp2=PCIN>>17  opr=+  inp1=P  carry=CIN  dbl_ovrd=off  block_type=constant
  dout : Outport
  of : Outport  Port=2
  wires:
  din/1 -> convert/1
  convert/1 -> dout/1
  never/1 -> of/1

== system casper_library_correlator/cross_multiplier/cvrt3_1_0_real ==
  din : Inport
  convert : casper_library_misc/convert  bin_pt_in=binary_point_i  n_bits_out=bit_width_o  bin_pt_out=binary_point_o  quantization=Truncate  overflow=Wrap  latency=latency
      settings: AttributesFormatString=|
      | N_7 ==> 4_3
      | truncate, wrap
      | latency = 4
  never : xbsIndex_r4/Constant  const=0  gui_display_data_type=Fixed-point  arith_type=Boolean  n_bits=16  bin_pt=14  preci_type=Single  exp_width=8  frac_width=24  explicit_period=on  period=1  equ=P=C  opselect=C  inp2=PCIN>>17  opr=+  inp1=P  carry=CIN  dbl_ovrd=off  block_type=constant
  dout : Outport
  of : Outport  Port=2
  wires:
  din/1 -> convert/1
  convert/1 -> dout/1
  never/1 -> of/1

== system casper_library_correlator/cross_multiplier/cvrt3_1_1_imag ==
  din : Inport
  convert : casper_library_misc/convert  bin_pt_in=binary_point_i  n_bits_out=bit_width_o  bin_pt_out=binary_point_o  quantization=Truncate  overflow=Wrap  latency=latency
      settings: AttributesFormatString=|
      | N_7 ==> 4_3
      | truncate, wrap
      | latency = 4
  never : xbsIndex_r4/Constant  const=0  gui_display_data_type=Fixed-point  arith_type=Boolean  n_bits=16  bin_pt=14  preci_type=Single  exp_width=8  frac_width=24  explicit_period=on  period=1  equ=P=C  opselect=C  inp2=PCIN>>17  opr=+  inp1=P  carry=CIN  dbl_ovrd=off  block_type=constant
  dout : Outport
  of : Outport  Port=2
  wires:
  din/1 -> convert/1
  convert/1 -> dout/1
  never/1 -> of/1

== system casper_library_correlator/cross_multiplier/cvrt3_1_1_real ==
  din : Inport
  convert : casper_library_misc/convert  bin_pt_in=binary_point_i  n_bits_out=bit_width_o  bin_pt_out=binary_point_o  quantization=Truncate  overflow=Wrap  latency=latency
      settings: AttributesFormatString=|
      | N_7 ==> 4_3
      | truncate, wrap
      | latency = 4
  never : xbsIndex_r4/Constant  const=0  gui_display_data_type=Fixed-point  arith_type=Boolean  n_bits=16  bin_pt=14  preci_type=Single  exp_width=8  frac_width=24  explicit_period=on  period=1  equ=P=C  opselect=C  inp2=PCIN>>17  opr=+  inp1=P  carry=CIN  dbl_ovrd=off  block_type=constant
  dout : Outport
  of : Outport  Port=2
  wires:
  din/1 -> convert/1
  convert/1 -> dout/1
  never/1 -> of/1

== system casper_library_correlator/cross_multiplier/cvrt3_2_0_imag ==
  din : Inport
  convert : casper_library_misc/convert  bin_pt_in=binary_point_i  n_bits_out=bit_width_o  bin_pt_out=binary_point_o  quantization=Truncate  overflow=Wrap  latency=latency
      settings: AttributesFormatString=|
      | N_7 ==> 4_3
      | truncate, wrap
      | latency = 4
  never : xbsIndex_r4/Constant  const=0  gui_display_data_type=Fixed-point  arith_type=Boolean  n_bits=16  bin_pt=14  preci_type=Single  exp_width=8  frac_width=24  explicit_period=on  period=1  equ=P=C  opselect=C  inp2=PCIN>>17  opr=+  inp1=P  carry=CIN  dbl_ovrd=off  block_type=constant
  dout : Outport
  of : Outport  Port=2
  wires:
  din/1 -> convert/1
  convert/1 -> dout/1
  never/1 -> of/1

== system casper_library_correlator/cross_multiplier/cvrt3_2_0_real ==
  din : Inport
  convert : casper_library_misc/convert  bin_pt_in=binary_point_i  n_bits_out=bit_width_o  bin_pt_out=binary_point_o  quantization=Truncate  overflow=Wrap  latency=latency
      settings: AttributesFormatString=|
      | N_7 ==> 4_3
      | truncate, wrap
      | latency = 4
  never : xbsIndex_r4/Constant  const=0  gui_display_data_type=Fixed-point  arith_type=Boolean  n_bits=16  bin_pt=14  preci_type=Single  exp_width=8  frac_width=24  explicit_period=on  period=1  equ=P=C  opselect=C  inp2=PCIN>>17  opr=+  inp1=P  carry=CIN  dbl_ovrd=off  block_type=constant
  dout : Outport
  of : Outport  Port=2
  wires:
  din/1 -> convert/1
  convert/1 -> dout/1
  never/1 -> of/1

== system casper_library_correlator/cross_multiplier/cvrt3_2_1_imag ==
  din : Inport
  convert : casper_library_misc/convert  bin_pt_in=binary_point_i  n_bits_out=bit_width_o  bin_pt_out=binary_point_o  quantization=Truncate  overflow=Wrap  latency=latency
      settings: AttributesFormatString=|
      | N_7 ==> 4_3
      | truncate, wrap
      | latency = 4
  never : xbsIndex_r4/Constant  const=0  gui_display_data_type=Fixed-point  arith_type=Boolean  n_bits=16  bin_pt=14  preci_type=Single  exp_width=8  frac_width=24  explicit_period=on  period=1  equ=P=C  opselect=C  inp2=PCIN>>17  opr=+  inp1=P  carry=CIN  dbl_ovrd=off  block_type=constant
  dout : Outport
  of : Outport  Port=2
  wires:
  din/1 -> convert/1
  convert/1 -> dout/1
  never/1 -> of/1

== system casper_library_correlator/cross_multiplier/cvrt3_2_1_real ==
  din : Inport
  convert : casper_library_misc/convert  bin_pt_in=binary_point_i  n_bits_out=bit_width_o  bin_pt_out=binary_point_o  quantization=Truncate  overflow=Wrap  latency=latency
      settings: AttributesFormatString=|
      | N_7 ==> 4_3
      | truncate, wrap
      | latency = 4
  never : xbsIndex_r4/Constant  const=0  gui_display_data_type=Fixed-point  arith_type=Boolean  n_bits=16  bin_pt=14  preci_type=Single  exp_width=8  frac_width=24  explicit_period=on  period=1  equ=P=C  opselect=C  inp2=PCIN>>17  opr=+  inp1=P  carry=CIN  dbl_ovrd=off  block_type=constant
  dout : Outport
  of : Outport  Port=2
  wires:
  din/1 -> convert/1
  convert/1 -> dout/1
  never/1 -> of/1

== system casper_library_correlator/cross_multiplier/cvrt3_3_0_imag ==
  din : Inport
  convert : casper_library_misc/convert  bin_pt_in=binary_point_i  n_bits_out=bit_width_o  bin_pt_out=binary_point_o  quantization=Truncate  overflow=Wrap  latency=latency
      settings: AttributesFormatString=|
      | N_7 ==> 4_3
      | truncate, wrap
      | latency = 4
  never : xbsIndex_r4/Constant  const=0  gui_display_data_type=Fixed-point  arith_type=Boolean  n_bits=16  bin_pt=14  preci_type=Single  exp_width=8  frac_width=24  explicit_period=on  period=1  equ=P=C  opselect=C  inp2=PCIN>>17  opr=+  inp1=P  carry=CIN  dbl_ovrd=off  block_type=constant
  dout : Outport
  of : Outport  Port=2
  wires:
  din/1 -> convert/1
  convert/1 -> dout/1
  never/1 -> of/1
